simulink model "r2_b8a4x128f_4gbe"  (R2012b)
(part 5 of 182)

  latch2/7(adc_over_reg) -> status2/7(out_adc_over)
  latch2/10(rx_bad_pkt_reg) -> status2/10(out_rx_bad_pkt)
  latch2/1(gbe_down_reg) -> status2/1(out_gbe_down)
  latch2/16(tx_reg) -> status2/16(out_txing_data)
  latch2/6(feng_chk_err_reg) -> status2/6(out_feng_chk_err)
  latch2/12(tx_over_reg) -> status2/12(out_tx_over)
  latch2/11(rx_bad_frame_reg) -> status2/11(out_rx_bad_frame)
  latch2/2(rx_dest_err_reg) -> status2/2(out_rx_dest_err)
  latch2/8(noise_diode_en_reg) -> status2/8(out_noise_diode_en)
  latch2/3(feng_rx_err_reg) -> status2/3(out_feng_rx_err)
  latch2/15(rx_reg) -> status2/15(out_rxing_data)
  latch2/5(feng_qdr_err_reg) -> status2/5(out_feng_qdr_err)
  latch2/4(fft_err_reg) -> status2/4(out_fft_err)
  latch2/9(vacc_err_reg) -> status2/9(out_vacc_err)
  latch2/13(xeng_bad_dat_reg) -> status2/13(out_xeng_bad_dat)
  latch2/17(data_bad) -> [data_in_bad2]
  latch2/18(error) -> [err2]
  latch2/19(flush_reg) -> status2/17(out_flushed)
  latch3/6(feng_chk_err_reg) -> status3/6(out_feng_chk_err)
  latch3/1(gbe_down_reg) -> status3/1(out_gbe_down)
  latch3/12(tx_over_reg) -> status3/12(out_tx_over)
  latch3/13(xeng_bad_dat_reg) -> status3/13(out_xeng_bad_dat)
  latch3/15(rx_reg) -> status3/15(out_rxing_data)
  latch3/7(adc_over_reg) -> status3/7(out_adc_over)
  latch3/8(noise_diode_en_reg) -> status3/8(out_noise_diode_en)
  latch3/11(rx_bad_frame_reg) -> status3/11(out_rx_bad_frame)
  latch3/16(tx_reg) -> status3/16(out_txing_data)
  latch3/10(rx_bad_pkt_reg) -> status3/10(out_rx_bad_pkt)
  latch3/9(vacc_err_reg) -> status3/9(out_vacc_err)
  latch3/3(feng_rx_err_reg) -> status3/3(out_feng_rx_err)
  latch3/14(pack_err_reg) -> status3/14(out_pack_err)
  latch3/4(fft_err_reg) -> status3/4(out_fft_err)
  latch3/5(feng_qdr_err_reg) -> status3/5(out_feng_qdr_err)
  latch3/2(rx_dest_err_reg) -> status3/2(out_rx_dest_err)
  latch3/17(data_bad) -> [data_in_bad3]
  latch3/19(flush_reg) -> status3/17(out_flushed)
  latch3/18(error) -> [err3]
  bus_expand2/1(msb_out5) -> [err_parity0]
  bus_expand2/2(out4) -> [err_output_of0]
  bus_expand2/3(out3) -> [err_rst0]
  bus_expand2/4(out2) -> [err_input_of0]
  bus_expand2/5(lsb_out1) -> [err_calfail0]
  bus_expand1/1(msb_out5) -> [err_parity1]
  bus_expand1/2(out4) -> [err_output_of1]
  bus_expand1/3(out3) -> [err_rst1]
  bus_expand1/4(out2) -> [err_input_of1]
  bus_expand1/5(lsb_out1) -> [err_calfail1]
  bus_expand9/1(msb_out5) -> [err_parity2]
  bus_expand9/2(out4) -> [err_output_of2]
  bus_expand9/3(out3) -> [err_rst2]
  bus_expand9/4(out2) -> [err_input_of2]
  bus_expand9/5(lsb_out1) -> [err_calfail2]
  bus_expand4/1(msb_out5) -> [err_parity3]
  bus_expand4/2(out4) -> [err_output_of3]
  bus_expand4/3(out3) -> [err_rst3]
  bus_expand4/4(out2) -> [err_input_of3]
  bus_expand4/5(lsb_out1) -> [err_calfail3]
  [pre_rx_dest_err0] -> Subsystem5/5(dest_err)
  Subsystem5/3(desterr_cnt) -> dest_err_cnt0/1(out_reg)
  [spead_error1] -> Subsystem2/4(flag)
  [spead_eof1] -> Subsystem2/3(eof)
  [spead_valid1] -> Subsystem2/2(we)
  Subsystem2/1(rx_cnt) -> rx_cnt1/1(out_reg)
  Subsystem2/2(err_cnt) -> rx_err_cnt1/1(out_reg)
  Subsystem2/3(desterr_cnt) -> dest_err_cnt1/1(out_reg)
  [pre_rx_dest_err1] -> Subsystem2/5(dest_err)
  gbe2/1(led_up) -> [gbe_up2]
  gbe2/2(led_rx) -> Terminator26/1
  gbe2/3(led_tx) -> Terminator6/1
  gbe2/4(tx_afull) -> Terminator8/1
  gbe2/5(tx_overflow) -> [gbe_tx_over2]
  gbe2/12(rx_overrun) -> Terminator12/1
  gbe2/11(rx_bad_frame) -> [gbe_rx_bad2]
  gbe2/6(rx_data) -> [gbe_rxdata2]
  gbe2/7(rx_valid) -> [gbe_rxvld2]
  gbe2/8(rx_source_ip) -> Terminator9/1
  gbe2/9(rx_source_port) -> Terminator10/1
  gbe2/10(rx_end_of_frame) -> [gbe_rxeof2]
  Constant4/1 -> gbe2/7(rx_ack)
  Constant5/1 -> gbe2/8(rx_overrun_ack)
  Constant6/1 -> gbe3/7(rx_ack)
  Constant3/1 -> gbe3/8(rx_overrun_ack)
  gbe3/11(rx_bad_frame) -> [gbe_rx_bad3]
  gbe3/5(tx_overflow) -> [gbe_tx_over3]
  gbe3/1(led_up) -> [gbe_up3]
  [gbe_debug_rst] -> gbe2/9(debug_rst)
  [gbe_debug_rst] -> gbe3/9(debug_rst)
  gbe3/2(led_rx) -> Terminator16/1
  gbe3/3(led_tx) -> Terminator20/1
  gbe3/4(tx_afull) -> Terminator21/1
  gbe3/8(rx_source_ip) -> Terminator22/1
  gbe3/9(rx_source_port) -> Terminator24/1
  gbe3/12(rx_overrun) -> Terminator25/1
  gbe3/6(rx_data) -> [gbe_rxdata3]
  gbe3/7(rx_valid) -> [gbe_rxvld3]
  gbe3/10(rx_end_of_frame) -> [gbe_rxeof3]
  [gbe_rst] -> gbe2/1(rst)
  [gbe_txd2] -> gbe2/2(tx_data)
  [gbe_txvld2] -> gbe2/3(tx_valid)
  [gbe_txip] -> gbe2/4(tx_dest_ip)
  [gbe_txport] -> gbe2/5(tx_dest_port)
  [gbe_txeof2] -> gbe2/6(tx_end_of_frame)
  [gbe_rst] -> gbe3/1(rst)
  [gbe_txd3] -> gbe3/2(tx_data)
  [gbe_txvld3] -> gbe3/3(tx_valid)
  [gbe_txip] -> gbe3/4(tx_dest_ip)
  [gbe_txport] -> gbe3/5(tx_dest_port)
  [gbe_txeof3] -> gbe3/6(tx_end_of_frame)
  Constant7/1 -> [gbe_txd2]
  Constant10/1 -> [gbe_txvld2]
  Constant11/1 -> [gbe_txeof2]
  Constant15/1 -> [gbe_txd3]
  Constant12/1 -> [gbe_txvld3]
  Constant14/1 -> [gbe_txeof3]
  [gbe_rxvld2] -> Delay41/1(d)
  [gbe_rxdata2] -> Delay40/1(d)
  [gbe_rxeof2] -> Delay42/1(d)
  Delay40/1(q) -> spead_unpack2/1(pkt_data)
  Delay41/1(q) -> spead_unpack2/2(pkt_valid)
  Delay42/1(q) -> spead_unpack2/3(pkt_eof)
  spead_unpack2/1(pkt_start) -> Terminator34/1
  spead_unpack2/2(data64) -> [spead_data2]
  spead_unpack2/3(valid64) -> [spead_valid2]
  spead_unpack2/4(eof64) -> [spead_eof2]
  spead_unpack2/5(error) -> [spead_error2]
  spead_unpack2/6(hdr_heap_id) -> Terminator29/1
  spead_unpack2/7(hdr_heap_size) -> Terminator30/1
  spead_unpack2/8(hdr_heap_offset) -> Terminator33/1
  spead_unpack2/9(hdr_pkt_len) -> Terminator27/1
  spead_unpack2/11(hdr6_0x4101_DIR) -> [spead_hdr2_2]
  spead_unpack2/12(hdr7_0x4102_DIR) -> [spead_hdr3_2]
  spead_unpack2/13(hdr8_0x4103_DIR) -> [spead_hdr4_2]
  spead_unpack2/14(hdr9_0x4300) -> Terminator37/1
  spead_unpack2/10(hdr5_0x1600_DIR) -> [spead_hdr1_2]
  [gbe_rxvld3] -> Delay44/1(d)
  [gbe_rxdata3] -> Delay43/1(d)
  [gbe_rxeof3] -> Delay45/1(d)
  Delay43/1(q) -> spead_unpack3/1(pkt_data)
  Delay44/1(q) -> spead_unpack3/2(pkt_valid)
  Delay45/1(q) -> spead_unpack3/3(pkt_eof)
  spead_unpack3/1(pkt_start) -> Terminator43/1
  spead_unpack3/2(data64) -> [spead_data3]
  spead_unpack3/3(valid64) -> [spead_valid3]
  spead_unpack3/4(eof64) -> [spead_eof3]
  spead_unpack3/5(error) -> [spead_error3]
  spead_unpack3/6(hdr_heap_id) -> Terminator40/1
  spead_unpack3/7(hdr_heap_size) -> Terminator41/1
  spead_unpack3/8(hdr_heap_offset) -> Terminator42/1
  spead_unpack3/9(hdr_pkt_len) -> Terminator39/1
  spead_unpack3/11(hdr6_0x4101_DIR) -> [spead_hdr2_3]
  spead_unpack3/12(hdr7_0x4102_DIR) -> [spead_hdr3_3]
  spead_unpack3/13(hdr8_0x4103_DIR) -> [spead_hdr4_3]
  spead_unpack3/14(hdr9_0x4300) -> Terminator44/1
  spead_unpack3/10(hdr5_0x1600_DIR) -> [spead_hdr1_3]
  [cnt_rst] -> Subsystem1/1(rst)
  [spead_error2] -> Subsystem1/4(flag)
  [spead_eof2] -> Subsystem1/3(eof)
  [spead_valid2] -> Subsystem1/2(we)
  Subsystem1/1(rx_cnt) -> rx_cnt2/1(out_reg)
  Subsystem1/2(err_cnt) -> rx_err_cnt2/1(out_reg)
  Subsystem1/3(desterr_cnt) -> dest_err_cnt2/1(out_reg)
  [pre_rx_dest_err2] -> Subsystem1/5(dest_err)
  [cnt_rst] -> Subsystem3/1(rst)
  [spead_error3] -> Subsystem3/4(flag)
  [spead_eof3] -> Subsystem3/3(eof)
  [spead_valid3] -> Subsystem3/2(we)
  Subsystem3/1(rx_cnt) -> rx_cnt3/1(out_reg)
  Subsystem3/2(err_cnt) -> rx_err_cnt3/1(out_reg)
  Subsystem3/3(desterr_cnt) -> dest_err_cnt3/1(out_reg)
  [pre_rx_dest_err3] -> Subsystem3/5(dest_err)
  bf_config/1(in_data_id) -> pipeline26/1(d)
  bf_config/2(in_time_id) -> pipeline27/1(d)
  bf0_config/2(in_beam_id) -> pipeline38/1(d)
  bf0_config/3(in_n_partitions) -> pipeline37/1(d)
  bf0_config/1(in_rst) -> pipeline36/1(d)
  bf0_partitions/1(in_partition0_offset) -> pipeline39/1(d)
  bf0_partitions/2(in_partition1_offset) -> pipeline40/1(d)
  bf0_partitions/3(in_partition2_offset) -> pipeline41/1(d)
  bf0_partitions/4(in_partition3_offset) -> pipeline42/1(d)
  bf1_partitions/1(in_partition0_offset) -> pipeline46/1(d)
  bf1_partitions/2(in_partition1_offset) -> pipeline47/1(d)
  bf1_partitions/3(in_partition2_offset) -> pipeline48/1(d)
  bf1_partitions/4(in_partition3_offset) -> pipeline49/1(d)
  bf_control/2(in_stream) -> pipeline29/1(d)
  bf_control/3(in_antenna) -> pipeline30/1(d)
  bf_control/1(in_beng) -> pipeline28/1(d)
  pipeline26/1(q) -> [bf_data_id]
  pipeline27/1(q) -> [bf_time_id]
  pipeline28/1(q) -> [bf_beng]
  pipeline29/1(q) -> [bf_stream]
  pipeline30/1(q) -> [bf_antenna]
  pipeline36/1(q) -> [bf0_rst]
  pipeline37/1(q) -> [bf0_n_partitions]
  pipeline38/1(q) -> Convert/1
  pipeline39/1(q) -> [bf0_partition_offset0]
  pipeline40/1(q) -> [bf0_partition_offset1]
  pipeline41/1(q) -> [bf0_partition_offset2]
  pipeline42/1(q) -> [bf0_partition_offset3]
  pipeline46/1(q) -> [bf1_partition_offset0]
  pipeline47/1(q) -> [bf1_partition_offset1]
  pipeline48/1(q) -> [bf1_partition_offset2]
  pipeline49/1(q) -> [bf1_partition_offset3]
  bf0_config/4(in_port) -> pipeline31/1(d)
  pipeline31/1(q) -> [bf0_txport]
  bf0_ip/1(in_ip) -> pipeline51/1(d)
  pipeline51/1(q) -> [bf0_txip]
  bf1_ip/1(in_ip) -> pipeline52/1(d)
  pipeline52/1(q) -> [bf1_txip]
  [cnt_rst] -> Subsystem/1(rst)
  [bf0s_eof0] -> Subsystem/2(of0)
  Subsystem/1(Out1) -> bf0_out_count/1(out_count0)
  [bf0s_eof2] -> Subsystem/4(of2)
  [bf0s_eof1] -> Subsystem/3(of1)
  [bf0s_eof3] -> Subsystem/5(of3)
  Subsystem/2(Out2) -> bf0_out_count/2(out_count1)
  Subsystem/3(Out3) -> bf0_out_count/3(out_count2)
  Subsystem/4(Out4) -> bf0_out_count/4(out_count3)
  [cnt_rst] -> Subsystem4/1(rst)
  [bf0s_of0] -> Subsystem4/2(of0)
  Subsystem4/1(Out1) -> bf0_of_count/1(out_count0)
  [bf0s_of2] -> Subsystem4/4(of2)
  [bf0s_of1] -> Subsystem4/3(of1)
  [bf0s_of3] -> Subsystem4/5(of3)
  Subsystem4/2(Out2) -> bf0_of_count/2(out_count1)
  Subsystem4/3(Out3) -> bf0_of_count/3(out_count2)
  Subsystem4/4(Out4) -> bf0_of_count/4(out_count3)
  pipeline53/1(q) -> [bf_value_filt]
  pipeline54/1(q) -> [bf_value_dupl]
  pipeline55/1(q) -> [bf_value_bw]
  pipeline56/1(q) -> [bf_value_quant]
  bf_value_in0/1(in_dupl) -> pipeline54/1(d)
  bf_value_in1/1(in_quant) -> pipeline56/1(d)
  bf_value_in1/2(in_filt) -> pipeline53/1(d)
  bf_value_ctrl/1(in_dupl) -> pipeline32/1(d)
  bf_value_ctrl/3(in_quant) -> pipeline34/1(d)
  pipeline32/1(q) -> edge_detect6/1
  pipeline33/1(q) -> edge_detect7/1
  pipeline34/1(q) -> edge_detect8/1
  pipeline57/1(q) -> edge_detect9/1
  bf_value_ctrl/2(in_bw) -> pipeline33/1(d)
  bf_value_ctrl/4(in_filt) -> pipeline57/1(d)
  bf_value_in0/2(in_bw) -> pipeline55/1(d)
  [bfout_valbw0] -> Delay27/1(d)
  [bfout_valquant0] -> Delay30/1(d)
  [bfout_valfilt0] -> Delay31/1(d)
  [bfout_valbw1] -> Delay26/1(d)
  [bfout_valbw2] -> Delay28/1(d)
  [bfout_valbw3] -> Delay32/1(d)
  [bfout_valquant1] -> Delay33/1(d)
  [bfout_valquant2] -> Delay35/1(d)
  [bfout_valquant3] -> Delay36/1(d)
  [bfout_valfilt1] -> Delay37/1(d)
  [bfout_valfilt2] -> Delay38/1(d)
  [bfout_valfilt3] -> Delay46/1(d)
  Delay27/1(q) -> bf_valout_bw0/1(out_bw0)
  Delay26/1(q) -> bf_valout_bw0/2(out_bw1)
  Delay32/1(q) -> bf_valout_bw1/2(out_bw3)
  Delay28/1(q) -> bf_valout_bw1/1(out_bw2)
  Delay30/1(q) -> bf_valout_quant0/1(out_quant0)
  Delay33/1(q) -> bf_valout_quant0/2(out_quant1)
  Delay36/1(q) -> bf_valout_quant1/2(out_quant3)
  Delay35/1(q) -> bf_valout_quant1/1(out_quant2)
  Delay37/1(q) -> bf_valout_filt/2(out_filt1)
  Delay38/1(q) -> bf_valout_filt/3(out_filt2)
  Delay46/1(q) -> bf_valout_filt/4(out_filt3)
  Delay31/1(q) -> bf_valout_filt/1(out_filt0)
  edge_detect6/1 -> [bf_valctrl_dupl]
  edge_detect7/1 -> [bf_valctrl_bw]
  edge_detect8/1 -> [bf_valctrl_quant]
  edge_detect9/1 -> [bf_valctrl_filt]
  [cnt_rst] -> Subsystem6/1(rst)
  [bf1s_eof0] -> Subsystem6/2(of0)
  Subsystem6/1(Out1) -> bf1_out_count/1(out_count0)
  [bf1s_eof2] -> Subsystem6/4(of2)
  [bf1s_eof1] -> Subsystem6/3(of1)
  [bf1s_eof3] -> Subsystem6/5(of3)
  Subsystem6/2(Out2) -> bf1_out_count/2(out_count1)
  Subsystem6/3(Out3) -> bf1_out_count/3(out_count2)
  Subsystem6/4(Out4) -> bf1_out_count/4(out_count3)
  [cnt_rst] -> Subsystem7/1(rst)
  [bf1s_of0] -> Subsystem7/2(of0)
  Subsystem7/1(Out1) -> bf1_of_count/1(out_count0)
  [bf1s_of2] -> Subsystem7/4(of2)
  [bf1s_of1] -> Subsystem7/3(of1)
  [bf1s_of3] -> Subsystem7/5(of3)
  Subsystem7/2(Out2) -> bf1_of_count/2(out_count1)
  Subsystem7/3(Out3) -> bf1_of_count/3(out_count2)
  Subsystem7/4(Out4) -> bf1_of_count/4(out_count3)
  pipeline35/1(q) -> [bf0_txen]
  bf0_config/5(in_txen) -> pipeline35/1(d)
  Convert/1 -> [bf0_id]
  bf1_config/2(in_beam_id) -> pipeline58/1(d)
  bf1_config/3(in_n_partitions) -> pipeline50/1(d)
  bf1_config/1(in_rst) -> pipeline45/1(d)
  pipeline45/1(q) -> [bf1_rst]
  pipeline50/1(q) -> [bf1_n_partitions]
  pipeline58/1(q) -> Convert1/1
  bf1_config/4(in_port) -> pipeline43/1(d)
  pipeline43/1(q) -> [bf1_txport]
  pipeline44/1(q) -> [bf1_txen]
  bf1_config/5(in_txen) -> pipeline44/1(d)
  Convert1/1 -> [bf1_id]
  Concat5/1 -> gbe_mux_bus0/1(di)
  [pack_txd1] -> Concat5/2
  [pack_txd0] -> Concat5/1
  Concat6/1 -> gbe_mux_bus0/2(validi)
  Concat7/1 -> gbe_mux_bus0/3(eofi)
  gbe_mux_bus0/5(start) -> Delay12/1, bus_expand/1(bus_in)
  Concat9/1 -> gbe_mux_bus0/4(drdy)
  Constant26/1 -> gbe_mux_bus0/5(transmit)
  gbe_mux_bus0/2(do) -> Delay13/1
  gbe_mux_bus0/3(valido) -> Delay14/1
  gbe_mux_bus0/4(eofo) -> Delay15/1
  gbe_mux_bus0/6(flush) -> [flush0]
  [bf0s_d0] -> Concat5/3
  [bf1s_d0] -> Concat5/4
  [pack_txvld0] -> Concat6/1
  [pack_txvld1] -> Concat6/2
  [bf0s_en0] -> Concat6/3
  [bf1s_en0] -> Concat6/4
  [bf0s_eof0] -> Concat7/3
  [bf1s_eof0] -> Concat7/4
  [pack_txeof0] -> Concat7/1
  [pack_txeof1] -> Concat7/2
  [bf0s_pkt_ready0] -> Concat9/3
  [bf1s_pkt_ready0] -> Concat9/4
  [pack_ready1] -> Concat9/2
  [pack_ready0] -> Concat9/1
  [bf0s_d1] -> Concat5/5
  [bf1s_d1] -> Concat5/6
  [bf0s_en1] -> Concat6/5
  [bf1s_en1] -> Concat6/6
  [bf0s_eof1] -> Concat7/5
  [bf1s_eof1] -> Concat7/6
  [bf0s_pkt_ready1] -> Concat9/5
  [bf1s_pkt_ready1] -> Concat9/6
  bus_expand/1(msb_out6) -> [go0]
  bus_expand/2(out5) -> [go1]
  bus_expand/3(out4) -> [bf0_tx_pkt0]
  bus_expand/4(out3) -> [bf1_tx_pkt0]
  bus_expand/5(out2) -> [bf0_tx_pkt1]
  bus_expand/6(lsb_out1) -> [bf1_tx_pkt1]
  Concat1/1 -> gbe_mux_bus1/1(di)
  Concat2/1 -> gbe_mux_bus1/2(validi)
  Concat3/1 -> gbe_mux_bus1/3(eofi)
  gbe_mux_bus1/5(start) -> bus_expand3/1(bus_in)
  Concat4/1 -> gbe_mux_bus1/4(drdy)
  Constant1/1 -> gbe_mux_bus1/5(transmit)
  gbe_mux_bus1/2(do) -> Delay24/1
  gbe_mux_bus1/4(eofo) -> Delay22/1
  gbe_mux_bus1/6(flush) -> [flush1]
  gbe_mux_bus1/3(valido) -> Delay23/1
  [pack_txd2] -> Concat1/1
  [pack_txd3] -> Concat1/2
  [pack_txvld2] -> Concat2/1
  [pack_txvld3] -> Concat2/2
  [pack_txeof2] -> Concat3/1
  [pack_txeof3] -> Concat3/2
  [pack_ready2] -> Concat4/1
  [pack_ready3] -> Concat4/2
  bus_expand3/1(msb_out6) -> [go2]
  bus_expand3/2(out5) -> [go3]
  [bf0s_d2] -> Concat1/3
  [bf1s_d2] -> Concat1/4
  [bf0s_d3] -> Concat1/5
  [bf1s_d3] -> Concat1/6
  [bf0s_en2] -> Concat2/3
  [bf1s_en2] -> Concat2/4
  [bf0s_en3] -> Concat2/5
  [bf1s_en3] -> Concat2/6
  [bf0s_eof2] -> Concat3/3
  [bf1s_eof2] -> Concat3/4
  [bf0s_eof3] -> Concat3/5
  [bf1s_eof3] -> Concat3/6
  [bf0s_pkt_ready2] -> Concat4/3
  [bf1s_pkt_ready2] -> Concat4/4
  [bf0s_pkt_ready3] -> Concat4/5
  [bf1s_pkt_ready3] -> Concat4/6
  bus_expand3/3(out4) -> [bf0_tx_pkt2]
  bus_expand3/4(out3) -> [bf1_tx_pkt2]
  bus_expand3/5(out2) -> [bf0_tx_pkt3]
  bus_expand3/6(lsb_out1) -> [bf1_tx_pkt3]
  Delay13/1 -> [gbe_txd0]
  Delay14/1 -> [gbe_txvld0]
  Delay15/1 -> [gbe_txeof0]
  [gbe_txip] -> Mux1/3, Mux1/2
  gbe_mux_bus0/1(input) -> Mux2/1, Delay11/1, Mux1/1
  [bf1_txip] -> Mux1/7, Mux1/5
  [bf0_txip] -> Mux1/6, Mux1/4
  [bf0_txport] -> Mux2/6, Mux2/4
  [bf1_txport] -> Mux2/7, Mux2/5
  [gbe_txport] -> Mux2/3, Mux2/2
  Mux2/1 -> [gbe_txport0]
  Delay22/1 -> [gbe_txeof1]
  Delay23/1 -> [gbe_txvld1]
  Delay24/1 -> [gbe_txd1]
  [gbe_txip] -> Mux3/2, Mux3/3
  gbe_mux_bus1/1(input) -> Mux4/1, Mux3/1
  [bf1_txip] -> Mux3/5, Mux3/7
  [bf0_txip] -> Mux3/4, Mux3/6
  [bf0_txport] -> Mux4/4, Mux4/6
  [bf1_txport] -> Mux4/7, Mux4/5
  [gbe_txport] -> Mux4/2, Mux4/3
  Mux3/1 -> [gbe_txip1]
  Mux4/1 -> [gbe_txport1]
  Delay11/1 -> [gbe_ipsel0]
  Delay12/1 -> [gbe_txstart0]
  Mux1/1 -> [gbe_txip0]
